simulink model "DDMR_PID_Simplified"  (R2024b)
settings: Solver=VariableStepAuto  StartTime=0.0  StopTime=150  RelTol=1e-3
values from neighbouring files (symbols this model uses):
  L_f = 0.2    [LQR.m]    (also in Track.m; Track2.m)
  line_width = 0.03    [LQR.m]    (also in Track.m; Track2.m)
  track_pts = [2*cos(linspace(0, 2*pi, 1000)'), 2*sin(linspace(0, 2*pi, 1000)').*cos(linspace(0, 2*pi, 1000)')]    [LQR.m]    (also in Track.m; Track2.m = [track_pts; segments{i}])
  W_spread = 0.15    [LQR.m]    (also in Track.m; Track2.m)
libraries: slpidlib x2, robotmobilelib x1
settings Model: Creator=moham  LastModifiedBy=moham

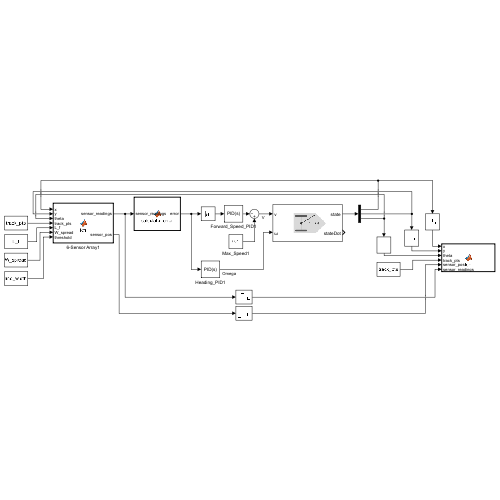
[thumbnail: Simulink's stored preview of the top-level diagram]
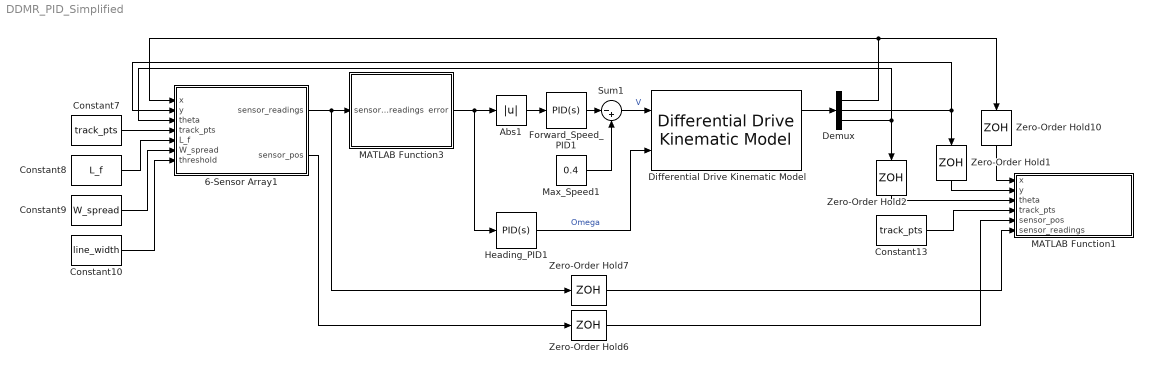
== system DDMR_PID_Simplified ==
  6-Sensor Array1 : MATLAB Function  TreatAsAtomicUnit=on
  Abs1 : Abs  SaturateOnIntegerOverflow=off
  Constant10 : Constant  Value=line_width
  Constant13 : Constant  Value=track_pts
  Constant7 : Constant  Value=track_pts
  Constant8 : Constant  Value=L_f
  Constant9 : Constant  Value=W_spread
  Demux : Demux  Outputs=3
  Differential Drive Kinematic Model : robotmobilelib/Differential Drive Kinematic Model  VehicleInputs=Vehicle Speed & Heading Angular Velocity  WheelRadius=R  WheelSpeedRange=[-inf inf]  TrackWidth=L  InitialState=[0; 0; pi/-3]  SimulateUsing=Code generation
  Forward_Speed_PID1 : slpidlib/PID Controller  Controller=PID  Form=Parallel  TimeDomain=Continuous-time  UseExternalTs=off  SampleTime=-1  IntegratorMethod=Forward Euler  FilterMethod=Forward Euler  ControllerParametersSource=internal  P=0.05  I=0  UseKiTs=off  D=0.01  UseExternalDerivativeSource=off  N=100  UseFilter=on  TunerSelectOption=Transfer Function Based (PID Tuner App)  InitialConditionSource=internal  InitialConditionForIntegrator=0  InitialConditionForFilter=0  DifferentiatorICPrevScaledInput=0  ExternalReset=none  TrackingMode=off  Kt=1  LimitOutput=off  SatLimitsSource=internal  UpperSaturationLimit=inf  LowerSaturationLimit=-inf  LinearizeAsGain=on  AntiWindupMode=none  Kb=1  LimitIntegrator=off  UpperIntegratorSaturationLimit=inf  LowerIntegratorSaturationLimit=-inf  POutMin=[]  POutMax=[]  IOutMin=[]  IOutMax=[]  DOutMin=[]  DOutMax=[]  NOutMin=[]  NOutMax=[]  SumOutMin=[]  SumOutMax=[]  SaturationOutMin=[]  SaturationOutMax=[]  PParamMin=[]  PParamMax=[]  IParamMin=[]  IParamMax=[]  DParamMin=[]  DParamMax=[]  NParamMin=[]  NParamMax=[]  KbParamMin=[]  KbParamMax=[]  KtParamMin=[]  KtParamMax=[]  KbOutMin=[]  KbOutMax=[]  KtOutMin=[]  KtOutMax=[]  IntegratorOutMin=[]  IntegratorOutMax=[]  FilterOutMin=[]  FilterOutMax=[]  SumI1OutMin=[]  SumI1OutMax=[]  SumI2OutMin=[]  SumI2OutMax=[]  SumI3OutMin=[]  SumI3OutMax=[]  SumI4OutMin=[]  SumI4OutMax=[]  SumDOutMin=[]  SumDOutMax=[]  DifferentiatorOutMin=[]  DifferentiatorOutMax=[]  FilterDiffOutCoefMin=[]  FilterDiffOutCoefMax=[]  ReciprocalOutMin=[]  ReciprocalOutMax=[]  SumDenOutMin=[]  SumDenOutMax=[]  SumNumOutMin=[]  SumNumOutMax=[]  DivideOutMin=[]  DivideOutMax=[]  UdiffTsProdOutMin=[]  UdiffTsProdOutMax=[]  NTsProdOutMin=[]  NTsProdOutMax=[]  UintegralTsProdOutMin=[]  UintegralTsProdOutMax=[]  UngainTsProdOutMin=[]  UngainTsProdOutMax=[]  ClampingZeroOutDataTypeStr=Inherit: Inherit via back propagation  ClampingZeroOutMin=[]  ClampingZeroOutMax=[]  FilterDenConstantOutDataTypeStr=Inherit: Inherit via back propagation  FilterDenConstantOutMin=[]  FilterDenConstantOutMax=[]  PCopyOutDataTypeStr=Inherit: Inherit via back propagation  PCopyOutMin=[]  PCopyOutMax=[]  NCopyOutDataTypeStr=Inherit: Inherit via back propagation  NCopyOutMin=[]  NCopyOutMax=[]  IntegratorContinuousStateAttributes=''  IntegratorStateMustResolveToSignalObject=off  IntegratorRTWStateStorageClass=Auto  FilterContinuousStateAttributes=''  FilterStateMustResolveToSignalObject=off  FilterRTWStateStorageClass=Auto  ParallelPVariant=InternalParameters  IdealPVariant=Disabled  IVariant=InternalParameters  DVariant=InternalParameters  IntegratorVariant=Continuous  SatVariant=Disabled  AWVariant=Passthrough  PCopyVariant=Disabled  TRVariant=Disabled  FdbkBlocksVariant=Forward  IdealPFdbkVariant=Disabled  SatFdbkVariant=Disabled  DerivativeFilterVariant=ContFilter  NVariant=InternalParameters  NCopyVariant=Disabled  FilterICVariant=InternalICsFilter  IntegratorICVariant=InternalICs  ExternalResetVariant=Disabled  TRSumVariant=Passthrough  SumFdbkVariant=Disabled  SumVariant=Sum_PID  TsampFilterVariant=InternalTs  TsampNgainVariant=Passthrough  TsampIntegralVariant=Disabled_SignalSpec  ExternalSaturationOutDataTypeStr=Inherit: Same as second input  DerivativeSourceVariant=ErrorSignal  PreIntVariant=InternalPreInt
  Heading_PID1 : slpidlib/PID Controller  Controller=PID  Form=Parallel  TimeDomain=Continuous-time  UseExternalTs=off  SampleTime=-1  IntegratorMethod=Forward Euler  FilterMethod=Forward Euler  ControllerParametersSource=internal  P=0.167  I=0.0001  UseKiTs=off  D=0.009  UseExternalDerivativeSource=off  N=100  UseFilter=on  TunerSelectOption=Transfer Function Based (PID Tuner App)  InitialConditionSource=internal  InitialConditionForIntegrator=0  InitialConditionForFilter=0  DifferentiatorICPrevScaledInput=0  ExternalReset=none  TrackingMode=off  Kt=1  LimitOutput=off  SatLimitsSource=internal  UpperSaturationLimit=inf  LowerSaturationLimit=-inf  LinearizeAsGain=on  AntiWindupMode=none  Kb=1  LimitIntegrator=off  UpperIntegratorSaturationLimit=inf  LowerIntegratorSaturationLimit=-inf  POutMin=[]  POutMax=[]  IOutMin=[]  IOutMax=[]  DOutMin=[]  DOutMax=[]  NOutMin=[]  NOutMax=[]  SumOutMin=[]  SumOutMax=[]  SaturationOutMin=[]  SaturationOutMax=[]  PParamMin=[]  PParamMax=[]  IParamMin=[]  IParamMax=[]  DParamMin=[]  DParamMax=[]  NParamMin=[]  NParamMax=[]  KbParamMin=[]  KbParamMax=[]  KtParamMin=[]  KtParamMax=[]  KbOutMin=[]  KbOutMax=[]  KtOutMin=[]  KtOutMax=[]  IntegratorOutMin=[]  IntegratorOutMax=[]  FilterOutMin=[]  FilterOutMax=[]  SumI1OutMin=[]  SumI1OutMax=[]  SumI2OutMin=[]  SumI2OutMax=[]  SumI3OutMin=[]  SumI3OutMax=[]  SumI4OutMin=[]  SumI4OutMax=[]  SumDOutMin=[]  SumDOutMax=[]  DifferentiatorOutMin=[]  DifferentiatorOutMax=[]  FilterDiffOutCoefMin=[]  FilterDiffOutCoefMax=[]  ReciprocalOutMin=[]  ReciprocalOutMax=[]  SumDenOutMin=[]  SumDenOutMax=[]  SumNumOutMin=[]  SumNumOutMax=[]  DivideOutMin=[]  DivideOutMax=[]  UdiffTsProdOutMin=[]  UdiffTsProdOutMax=[]  NTsProdOutMin=[]  NTsProdOutMax=[]  UintegralTsProdOutMin=[]  UintegralTsProdOutMax=[]  UngainTsProdOutMin=[]  UngainTsProdOutMax=[]  ClampingZeroOutDataTypeStr=Inherit: Inherit via back propagation  ClampingZeroOutMin=[]  ClampingZeroOutMax=[]  FilterDenConstantOutDataTypeStr=Inherit: Inherit via back propagation  FilterDenConstantOutMin=[]  FilterDenConstantOutMax=[]  PCopyOutDataTypeStr=Inherit: Inherit via back propagation  PCopyOutMin=[]  PCopyOutMax=[]  NCopyOutDataTypeStr=Inherit: Inherit via back propagation  NCopyOutMin=[]  NCopyOutMax=[]  IntegratorContinuousStateAttributes=''  IntegratorStateMustResolveToSignalObject=off  IntegratorRTWStateStorageClass=Auto  FilterContinuousStateAttributes=''  FilterStateMustResolveToSignalObject=off  FilterRTWStateStorageClass=Auto  ParallelPVariant=InternalParameters  IdealPVariant=Disabled  IVariant=InternalParameters  DVariant=InternalParameters  IntegratorVariant=Continuous  SatVariant=Disabled  AWVariant=Passthrough  PCopyVariant=Disabled  TRVariant=Disabled  FdbkBlocksVariant=Forward  IdealPFdbkVariant=Disabled  SatFdbkVariant=Disabled  DerivativeFilterVariant=ContFilter  NVariant=InternalParameters  NCopyVariant=Disabled  FilterICVariant=InternalICsFilter  IntegratorICVariant=InternalICs  ExternalResetVariant=Disabled  TRSumVariant=Passthrough  SumFdbkVariant=Disabled  SumVariant=Sum_PID  TsampFilterVariant=InternalTs  TsampNgainVariant=Passthrough  TsampIntegralVariant=Disabled_SignalSpec  ExternalSaturationOutDataTypeStr=Inherit: Same as second input  DerivativeSourceVariant=ErrorSignal  PreIntVariant=InternalPreInt
  MATLAB Function1 : MATLAB Function  TreatAsAtomicUnit=on
  MATLAB Function3 : MATLAB Function  TreatAsAtomicUnit=on
  Max_Speed1 : Constant  Value=0.4
  Sum1 : Sum  Inputs=|-+
  Zero-Order Hold{1..2,6..7,10} (5 alike) : ZeroOrderHold  SampleTime=0.033
  wires:
  Demux/2 -> Zero-Order Hold1/1, 6-Sensor Array1/2(y)
  Demux/1 -> Zero-Order Hold10/1, 6-Sensor Array1/1(x)
  Constant13/1 -> MATLAB Function1/4(track_pts)
  Zero-Order Hold7/1 -> MATLAB Function1/6(sensor_readings)
  6-Sensor Array1/1(sensor_readings) -> Zero-Order Hold7/1, MATLAB Function3/1(sensor_readings)
  Constant8/1 -> 6-Sensor Array1/5(L_f)
  Zero-Order Hold6/1 -> MATLAB Function1/5(sensor_pos)
  Constant7/1 -> 6-Sensor Array1/4(track_pts)
  MATLAB Function3/1(error) -> Heading_PID1/1, Abs1/1
  Sum1/1 -> Differential Drive Kinematic Model/1  "V"
  Constant9/1 -> 6-Sensor Array1/6(W_spread)
  Constant10/1 -> 6-Sensor Array1/7(threshold)
  6-Sensor Array1/2(sensor_pos) -> Zero-Order Hold6/1
  Forward_Speed_PID1/1 -> Sum1/1
  Heading_PID1/1 -> Differential Drive Kinematic Model/2  "Omega"
  Abs1/1 -> Forward_Speed_PID1/1
  Demux/3 -> Zero-Order Hold2/1, 6-Sensor Array1/3(theta)
  Differential Drive Kinematic Model/1 -> Demux/1
  Max_Speed1/1 -> Sum1/2
  Zero-Order Hold10/1 -> MATLAB Function1/1(x)
  Zero-Order Hold1/1 -> MATLAB Function1/2(y)
  Zero-Order Hold2/1 -> MATLAB Function1/3(theta)

== matlab function DDMR_PID_Simplified/6-Sensor Array1 ==
  data: x input; sensor_readings output; y input; theta input; track_pts input; L_f input; W_spread input; threshold input; sensor_pos output
function [sensor_readings, sensor_pos] = fcn(x, y, theta, track_pts, L_f, W_spread, threshold)
    % 6 sensors spread linearly across the front
    y_offsets = linspace(W_spread/2, -W_spread/2, 6);
    S_loc = [L_f * ones(1,6); y_offsets];
    
    R = [cos(theta), -sin(theta); sin(theta), cos(theta)];
    
    sensor_pos = zeros(2, 6);
    sensor_readings = zeros(1, 6);
    
    for i = 1:6
        % Calculate global position of each sensor
        sensor_pos(:, i) = [x; y] + R * S_loc(:, i);
        
        % Check distance to the track
        dists = sqrt((track_pts(:,1) - sensor_pos(1, i)).^2 + (track_pts(:,2) - sensor_pos(2, i)).^2);
        if min(dists) <= threshold
            sensor_readings(i) = 1;
        end
    end
end

== matlab function DDMR_PID_Simplified/MATLAB Function1 ==
  settings: updateMethod=DISCRETE
  data: x input; y input; theta input; track_pts input; sensor_pos input; sensor_readings input
function fcn(x, y, theta, track_pts, sensor_pos, sensor_readings)
    coder.extrinsic('figure', 'plot', 'hold', 'scatter', 'drawnow', 'gca', 'cla', 'axis', 'grid', 'ishandle', 'xlim', 'ylim');
    
    persistent fig;
    
    if isempty(fig)
        fig = figure('Name', '6-Sensor DDMR');
    elseif ~ishandle(fig)
        fig = figure('Name', '6-Sensor DDMR');
    end
    
    figure(fig); 
    ax = gca; 
    cla(ax); 
    hold(ax, 'on');
    
    % Draw Track
    plot(ax, track_pts(:,1), track_pts(:,2), 'k--', 'LineWidth', 2);
    
    % Draw Robot (Scaled to fit your L = 0.2m physical track width)
    R_chassis = 0.12; 
    th = linspace(0, 2*pi, 50);
    plot(ax, x + R_chassis*cos(th), y + R_chassis*sin(th), 'b', 'LineWidth', 1.5);
    
    % Plot heading line (Starts at the chassis edge, extends past the sensors to 0.3m)
    Pointer_L = 0.3; 
    plot(ax, [x + R_chassis*cos(theta), x + Pointer_L*cos(theta)], ...
             [y + R_chassis*sin(theta), y + Pointer_L*sin(theta)], 'r', 'LineWidth', 2);
    
    % Draw 6 Sensors (Red = off line, Green = on line)
    for i = 1:6
        c = 'r'; 
        if sensor_readings(i) == 1
            c = 'g'; 
        end
        scatter(ax, sensor_pos(1, i), sensor_pos(2, i), 40, c, 'filled');
    end
    
    % Dynamic sliding camera fix
    axis(ax, 'equal'); 
    xlim(ax, [x - 0.8, x + 0.8]);
    ylim(ax, [y - 0.8, y + 0.8]);
    
    grid(ax, 'on'); 
    hold(ax, 'off'); 
    drawnow;
end

== matlab function DDMR_PID_Simplified/MATLAB Function3 ==
  settings: updateMethod=DISCRETE
  data: sensor_readings input; error output
function error = calculate_error(sensor_readings)
    % Assign weights to the 6 sensors: far left is positive error, far right is negative
    weights = [5, 3, 1, -1, -3, -5]; 
    
    % Multiply readings by weights and sum them up
    error = sum(sensor_readings .* weights);
    
    % If no line is detected, keep the previous error (prevents erratic spinning)
    persistent prev_error;
    if isempty(prev_error)
        prev_error = 0;
    end
    
  if sum(sensor_readings) == 0
    error = 0; % Command the robot to drive straight to re-intersect the track
else
    error = sum(sensor_readings .* weights);
end
